simulink subsystem "unreal_cosim"  (R2026a)
settings: Solver=VariableStepAuto
undefined symbols (not defined in the file): M_WorldToUCS, S, scene_config, Sim3dSensor
libraries: sim3dlib x32, visionsinks x4, sim3dcameralib x4, dspvision x4
PreSaveFcn:
  | deconfigure_scene(bdroot)
  | defaultToFileBlockNames(bdroot);
settings Model: Creator=kjhaydon  LastModifiedBy=kjhaydon

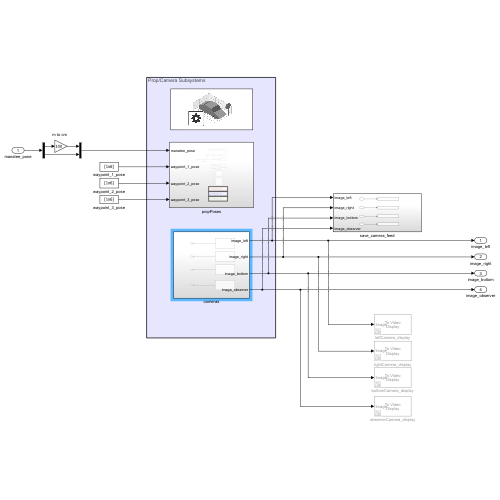
[thumbnail: Simulink's stored preview of the top-level diagram]
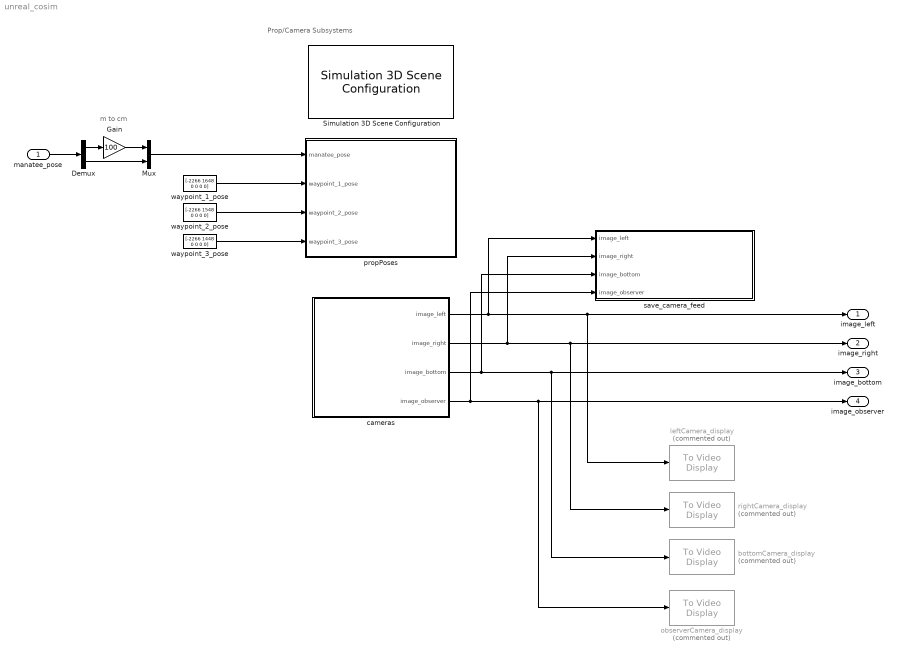
== system unreal_cosim ==
  note: m to cm
  note: Prop/Camera Subsystems
  manatee_pose : Inport  SampleTime=S.dt_sample
  Demux : Demux  Outputs=2
  Gain : Gain  Gain=100
  Mux : Mux  Inputs=2
  Simulation 3D Scene Configuration : sim3dlib/Simulation 3D Scene Configuration  Priority=0  ProjectFormat=Unreal Executable  SceneDesc=Empty scene  ProjectName=C:\Users\kjhaydon\Documents\GitHub\controls-2027\src\unreal_executables\EllingtonPoolSim_2_beta\Windows\EllingtonPoolSim2.exe  ScenePath=/Game/Olympic_Pool_Course  UEProjPath=C:\Users\Liam\OneDrive\Documents\Unreal Projects\EllingtonPoolSim2\EllingtonPoolSim2.uproject  EnableOpenDRIVE=off  vehTagList={'Custom';'Scene Origin'}  vehTag=Scene Origin  AttachedCameraRelativeTranslation=[0 0 0]  FreeCameraDefaultInitialTranslation=[-6, 0, 2]  AttachedCameraRelativeRotation=[0, -15, 0]  FreeCameraDefaultInitialRotation=[0, -15, 0]  ViewpointName=Custom  FreeCameraInitialTranslation=[0, 0, 0]  FreeCameraInitialRotation=[0, 0, 0]  OpVisEn=off  Ts=S.dt_sample  EnableWindow=off  EnableRemoteAccess=off  SimulationMode=CoSimulation  SimulateUsing=Interpreted execution  EnableAnimationRecording=off  OverrideDefaultRecording=off  AnimationRecordingFileName=sim3dAnimation.mat  AnimationRecordingInterval=[0 inf]  EnableWeather=off  SunAzimuth=90  SunAltitude=40.0  EnableGeospatialSun=off  Latitude=0  Longitude=0  Date=2023-01-01  Time=10:30:00  GeoTimeZone=-5.0  SunDaylightSaving=off  wind=1  clouds=10  EnableVolumetricClouds=off  CloudCoverage=0  CloudAltitude=6  fog=0  rain=0  RaindropsEffect=off  SnowDensity=0  EnableGeospatial=off  TilesetSource=Earth terrain  UseTrueOrigin=off  OriginHeight=200  OriginLatitude=40.744652  OriginLongitude=-73.988864  MapStyle=Aerial  AdditionalAssetIDs=[]  UseAdvancedSunSky=off  SolarTime=11  TimeZone=-5  Day=21  Month=9  Year=2022  UseDaylightSavingTime=on  DSTStartDay=10  DSTStartMonth=3  DSTEndDay=3  DSTEndMonth=11  DSTSwitchHour=2  sensorTag=MainCamera2  sensorId=2  sensorName=MainCamera2  mountLoc=Origin  offsetFlag=off  tmountOffset=[0, 0, 0]  rmountOffset=[0, 0, 0]  HorizontalResolution=1280  VerticalResolution=720  HorizontalFOV=60  mountPoint=[0 0 0]  mountOrientation=[0 0 0]  aMode=5  ID=2  GeoTrigger=Inactive  ViewNameList={'Custom'}  ViewTranslationList={'[0 0 0]'}  ViewRotationList={'[0 0 0]'}
      settings: LibrarySourceBlock=sl3dlib/Simulation 3D/Environment/Simulation 3D Scene Configuration
  bottomCamera_display : visionsinks/To Video Display  Commented=on  windowSizeMode=Normal  openAtMdlStart=off  fullScreen=off  videoWindowX=536805376  videoWindowY=536805376  saveWindowSize=off  videoWindowWidth=1491  videoWindowHeight=834  inputColorFormat=RGB  inputType=Obsolete  imagePorts=One multidimensional signal  OutputDevice=On-screen video monitor  dataOrg=Column-major  isWindowOpen=off
  cameras : Subsystem
  leftCamera_display : visionsinks/To Video Display  Commented=on  windowSizeMode=Normal  openAtMdlStart=on  fullScreen=off  videoWindowX=536805376  videoWindowY=536805376  saveWindowSize=off  videoWindowWidth=1491  videoWindowHeight=834  inputColorFormat=RGB  inputType=Obsolete  imagePorts=One multidimensional signal  OutputDevice=On-screen video monitor  dataOrg=Column-major  isWindowOpen=off
  observerCamera_display : visionsinks/To Video Display  Commented=on  windowSizeMode=Normal  openAtMdlStart=on  fullScreen=off  videoWindowX=536805376  videoWindowY=536805376  saveWindowSize=off  videoWindowWidth=1491  videoWindowHeight=834  inputColorFormat=RGB  inputType=Obsolete  imagePorts=One multidimensional signal  OutputDevice=On-screen video monitor  dataOrg=Column-major  isWindowOpen=off
  propPoses : Subsystem  Priority=1
  rightCamera_display : visionsinks/To Video Display  Commented=on  windowSizeMode=Normal  openAtMdlStart=on  fullScreen=off  videoWindowX=536805376  videoWindowY=536805376  saveWindowSize=off  videoWindowWidth=1491  videoWindowHeight=834  inputColorFormat=RGB  inputType=Obsolete  imagePorts=One multidimensional signal  OutputDevice=On-screen video monitor  dataOrg=Column-major  isWindowOpen=off
  save_camera_feed : Subsystem
  waypoint_1_pose : Constant  Value=[-2266 1648 0 0 0 0]
  waypoint_2_pose : Constant  Value=[-2266 1548 0 0 0 0]
  waypoint_3_pose : Constant  Value=[-2266 1448 0 0 0 0]
  image_left : Outport
  image_right : Outport  Port=2
  image_bottom : Outport  Port=3
  image_observer : Outport  Port=4
  wires:
  waypoint_3_pose/1 -> propPoses/4(waypoint_3_pose)
  waypoint_2_pose/1 -> propPoses/3(waypoint_2_pose)
  waypoint_1_pose/1 -> propPoses/2(waypoint_1_pose)
  Demux/1 -> Gain/1
  Gain/1 -> Mux/1
  Demux/2 -> Mux/2
  manatee_pose/1 -> Demux/1
  Mux/1 -> propPoses/1(manatee_pose)
  cameras/4(image_observer) -> save_camera_feed/4(image_observer), observerCamera_display/1, image_observer/1
  cameras/1(image_left) -> save_camera_feed/1(image_left), leftCamera_display/1, image_left/1
  cameras/2(image_right) -> rightCamera_display/1, image_right/1, save_camera_feed/2(image_right)
  cameras/3(image_bottom) -> bottomCamera_display/1, image_bottom/1, save_camera_feed/3(image_bottom)

== system unreal_cosim/cameras ==
  Bottom Camera ID:1 : sim3dcameralib/Simulation 3D Camera  Priority=1  sensorTag=Sim3dSensor�  sensorId=1  sensorName=Sim3dSensor�  vehTagList={'Custom ...';'Scene Origin'}  vehTag=Scene Origin  CoordinateSystem=Default  mountLoc=Origin  offsetFlag=on  tmountOffset=scene_config.cameras.bottomCamera.Position  extTmount=off  rmountOffset=scene_config.cameras.bottomCamera.Orientation  extRmount=off  FocalLength=scene_config.cameras.bottomCamera.FocalLength  OpticalCenter=scene_config.cameras.bottomCamera.OpticalCenter  ImageSize=scene_config.cameras.bottomCamera.ImageSize  RadialDistortion=scene_config.cameras.bottomCamera.RadialDistortion  TangentialDistortion=scene_config.cameras.bottomCamera.TangentialDistortion  SensorSkew=0  VisualizeFieldOfView=off  FieldOfViewRange=61  DepthOutportEnabled=off  SemanticOutportEnabled=off  TransformOutportEnabled=off  SampleTime=S.dt_sample  mountPoint=[0.23 0 -0.08]  mountOrientation=[0 -90 0]  aMode=5  ID=1
      settings: LibrarySourceBlock=sl3dlib/Simulation 3D/Sensors/Simulation 3D Camera
  Left Camera ID:2 : sim3dcameralib/Simulation 3D Camera  Priority=1  sensorTag=Sim3dSensor�  sensorId=2  sensorName=Sim3dSensor�  vehTagList={'Custom ...';'Scene Origin'}  vehTag=Scene Origin  CoordinateSystem=Default  mountLoc=Origin  offsetFlag=on  tmountOffset=scene_config.cameras.leftCamera.Position  extTmount=off  rmountOffset=scene_config.cameras.leftCamera.Orientation  extRmount=off  FocalLength=scene_config.cameras.leftCamera.FocalLength  OpticalCenter=scene_config.cameras.leftCamera.OpticalCenter  ImageSize=scene_config.cameras.leftCamera.ImageSize  RadialDistortion=scene_config.cameras.leftCamera.RadialDistortion  TangentialDistortion=scene_config.cameras.leftCamera.TangentialDistortion  SensorSkew=0  VisualizeFieldOfView=off  FieldOfViewRange=61  DepthOutportEnabled=off  SemanticOutportEnabled=off  TransformOutportEnabled=off  SampleTime=S.dt_sample  mountPoint=[0.38 -0.024 0.14]  mountOrientation=[0 0 0]  aMode=5  ID=2
      settings: LibrarySourceBlock=sl3dlib/Simulation 3D/Sensors/Simulation 3D Camera
  Observer Camera ID:4 : sim3dcameralib/Simulation 3D Camera  Priority=1  sensorTag=Sim3dSensor�  sensorId=4  sensorName=Sim3dSensor�  vehTagList={'Custom ...';'Scene Origin'}  vehTag=Scene Origin  CoordinateSystem=Default  mountLoc=Origin  offsetFlag=on  tmountOffset=scene_config.cameras.observerCamera.Position  extTmount=off  rmountOffset=scene_config.cameras.observerCamera.Orientation  extRmount=off  FocalLength=scene_config.cameras.observerCamera.FocalLength  OpticalCenter=scene_config.cameras.observerCamera.OpticalCenter  ImageSize=scene_config.cameras.observerCamera.ImageSize  RadialDistortion=scene_config.cameras.observerCamera.RadialDistortion  TangentialDistortion=scene_config.cameras.observerCamera.TangentialDistortion  SensorSkew=0  VisualizeFieldOfView=off  FieldOfViewRange=61  DepthOutportEnabled=off  SemanticOutportEnabled=off  TransformOutportEnabled=off  SampleTime=S.dt_sample  mountPoint=[0 0 0]  mountOrientation=[0 0 0]  aMode=5  ID=4
      settings: LibrarySourceBlock=sl3dlib/Simulation 3D/Sensors/Simulation 3D Camera
  Right Camera ID:3 : sim3dcameralib/Simulation 3D Camera  Priority=1  sensorTag=Sim3dSensor�  sensorId=3  sensorName=Sim3dSensor�  vehTagList={'Custom ...';'Scene Origin'}  vehTag=Scene Origin  CoordinateSystem=Default  mountLoc=Origin  offsetFlag=on  tmountOffset=scene_config.cameras.rightCamera.Position  extTmount=off  rmountOffset=scene_config.cameras.rightCamera.Orientation  extRmount=off  FocalLength=scene_config.cameras.rightCamera.FocalLength  OpticalCenter=scene_config.cameras.rightCamera.OpticalCenter  ImageSize=scene_config.cameras.rightCamera.ImageSize  RadialDistortion=scene_config.cameras.rightCamera.RadialDistortion  TangentialDistortion=scene_config.cameras.rightCamera.TangentialDistortion  SensorSkew=0  VisualizeFieldOfView=off  FieldOfViewRange=61  DepthOutportEnabled=off  SemanticOutportEnabled=off  TransformOutportEnabled=off  SampleTime=S.dt_sample  mountPoint=[0.38 0.024 0.14]  mountOrientation=[0 0 0]  aMode=5  ID=3
      settings: LibrarySourceBlock=sl3dlib/Simulation 3D/Sensors/Simulation 3D Camera
  image_left : Outport
  image_right : Outport  Port=2
  image_bottom : Outport  Port=3
  image_observer : Outport  Port=4
  wires:
  Observer Camera ID:4/1 -> image_observer/1
  Bottom Camera ID:1/1 -> image_bottom/1
  Right Camera ID:3/1 -> image_right/1
  Left Camera ID:2/1 -> image_left/1

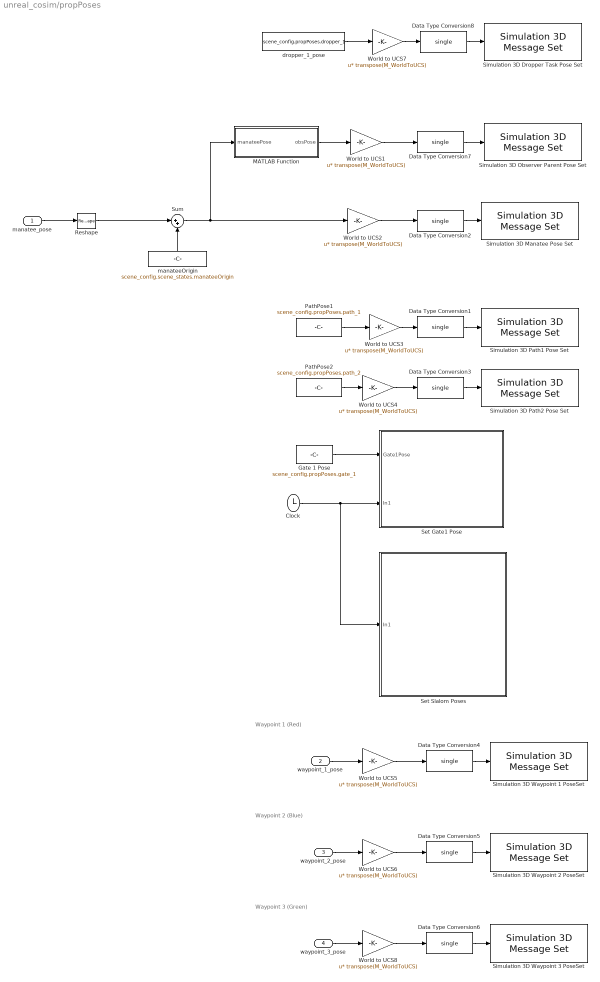
== system unreal_cosim/propPoses ==
  note: Waypoint 3 (Green)
  note: Waypoint 2 (Blue)
  note: Waypoint 1 (Red)
  manatee_pose : Inport
  waypoint_1_pose : Inport  Port=2
  waypoint_2_pose : Inport  Port=3
  waypoint_3_pose : Inport  Port=4
  Clock : Clock
      settings: Decimation=S.dt_sample/S.dt_sim
  Data Type Conversion{1..8} (8 alike) : DataTypeConversion  OutDataTypeStr=single  SaturateOnIntegerOverflow=off  RndMeth=Floor
  Gate 1 Pose : Constant  Value=scene_config.propPoses.gate_1
  MATLAB Function : MATLAB Function  TreatAsAtomicUnit=on
  PathPose1 : Constant  Value=scene_config.propPoses.path_1
  PathPose2 : Constant  Value=scene_config.propPoses.path_2
  Reshape : Reshape  OutputDimensionality=Row vector (2-D)
  Set Gate1 Pose : Subsystem
  Set Slalom Poses : Subsystem
  Simulation 3D Dropper Task Pose Set : sim3dlib/Simulation 3D Message Set  Priority=-1  SigName=DropperTask1PoseSet  Ts=S.dt_sample  aMode=0
      settings: LibrarySourceBlock=aerolibsim3d/Simulation 3D Message Set
  Simulation 3D Manatee Pose Set : sim3dlib/Simulation 3D Message Set  Priority=-1  SigName=ManateePoseSet  Ts=S.dt_sample  aMode=0
      settings: LibrarySourceBlock=aerolibsim3d/Simulation 3D Message Set
  Simulation 3D Observer Parent Pose Set : sim3dlib/Simulation 3D Message Set  Priority=-1  SigName=ParentPoseSet  Ts=S.dt_sample  aMode=0
      settings: LibrarySourceBlock=aerolibsim3d/Simulation 3D Message Set
  Simulation 3D Path1 Pose Set : sim3dlib/Simulation 3D Message Set  Priority=-1  SigName=Path1PoseSet  Ts=S.dt_sample  aMode=0
      settings: LibrarySourceBlock=aerolibsim3d/Simulation 3D Message Set
  Simulation 3D Path2 Pose Set : sim3dlib/Simulation 3D Message Set  Priority=-1  SigName=Path2PoseSet  Ts=S.dt_sample  aMode=0
      settings: LibrarySourceBlock=aerolibsim3d/Simulation 3D Message Set
  Simulation 3D Waypoint 1 PoseSet : sim3dlib/Simulation 3D Message Set  Priority=-1  SigName=Waypoint1PoseSet  Ts=S.dt_sample  aMode=0
      settings: LibrarySourceBlock=aerolibsim3d/Simulation 3D Message Set
  Simulation 3D Waypoint 2 PoseSet : sim3dlib/Simulation 3D Message Set  Priority=-1  SigName=Waypoint2PoseSet  Ts=S.dt_sample  aMode=0
      settings: LibrarySourceBlock=aerolibsim3d/Simulation 3D Message Set
  Simulation 3D Waypoint 3 PoseSet : sim3dlib/Simulation 3D Message Set  Priority=-1  SigName=Waypoint3PoseSet  Ts=S.dt_sample  aMode=0
      settings: LibrarySourceBlock=aerolibsim3d/Simulation 3D Message Set
  Sum : Sum  Inputs=|++
  World to UCS{1..8} (8 alike) : Gain  Gain=transpose(M_WorldToUCS)  Multiplication=Matrix(u*K)
  dropper_1_pose : Constant  Value=scene_config.propPoses.dropper_1
  manateeOrigin : Constant  Value=scene_config.scene_states.manateeOrigin
  wires:
  Reshape/1 -> Sum/1
  waypoint_3_pose/1 -> World to UCS8/1
  dropper_1_pose/1 -> World to UCS7/1
  World to UCS7/1 -> Data Type Conversion8/1
  Data Type Conversion8/1 -> Simulation 3D Dropper Task Pose Set/1
  MATLAB Function/1(obsPose) -> World to UCS1/1
  World to UCS1/1 -> Data Type Conversion7/1
  Data Type Conversion7/1 -> Simulation 3D Observer Parent Pose Set/1
  manateeOrigin/1 -> Sum/2
  Sum/1 -> MATLAB Function/1(manateePose), World to UCS2/1
  manatee_pose/1 -> Reshape/1
  Data Type Conversion6/1 -> Simulation 3D Waypoint 3 PoseSet/1
  World to UCS8/1 -> Data Type Conversion6/1
  World to UCS6/1 -> Data Type Conversion5/1
  Data Type Conversion5/1 -> Simulation 3D Waypoint 2 PoseSet/1
  waypoint_2_pose/1 -> World to UCS6/1
  World to UCS5/1 -> Data Type Conversion4/1
  Data Type Conversion4/1 -> Simulation 3D Waypoint 1 PoseSet/1
  waypoint_1_pose/1 -> World to UCS5/1
  World to UCS2/1 -> Data Type Conversion2/1
  Clock/1 -> Set Gate1 Pose/2(In1), Set Slalom Poses/1(In1)
  PathPose2/1 -> World to UCS4/1
  Data Type Conversion3/1 -> Simulation 3D Path2 Pose Set/1
  World to UCS4/1 -> Data Type Conversion3/1
  PathPose1/1 -> World to UCS3/1
  Data Type Conversion1/1 -> Simulation 3D Path1 Pose Set/1
  World to UCS3/1 -> Data Type Conversion1/1
  Data Type Conversion2/1 -> Simulation 3D Manatee Pose Set/1
  Gate 1 Pose/1 -> Set Gate1 Pose/1(Gate1Pose)

== system unreal_cosim/save_camera_feed ==
  image_left : Inport
  image_right : Inport  Port=2
  image_bottom : Inport  Port=3
  image_observer : Inport  Port=4
  bottomCamera_save : dspvision/To Multimedia File  Commented=on  outputFilename=default  streamSelection=Video only  videoCompressor=None (uncompressed)  audioCompressor=None (uncompressed)  imagePorts=One multidimensional signal  fileType=MPEG4  audioDatatype=16-bit integer  fourcc=RGB  audioBitRate=128  audioQuality=75  videoQuality=75  mj2000CompFactor=10
      settings: LibrarySourceBlock=audiosinks/To Multimedia File
  leftCamera_save : dspvision/To Multimedia File  Commented=on  outputFilename=default  streamSelection=Video only  videoCompressor=None (uncompressed)  audioCompressor=None (uncompressed)  imagePorts=One multidimensional signal  fileType=MPEG4  audioDatatype=16-bit integer  fourcc=RGB  audioBitRate=128  audioQuality=75  videoQuality=75  mj2000CompFactor=10
      settings: LibrarySourceBlock=audiosinks/To Multimedia File
  observerCamera_save : dspvision/To Multimedia File  Commented=on  outputFilename=default  streamSelection=Video only  videoCompressor=None (uncompressed)  audioCompressor=None (uncompressed)  imagePorts=One multidimensional signal  fileType=MPEG4  audioDatatype=16-bit integer  fourcc=RGB  audioBitRate=128  audioQuality=75  videoQuality=75  mj2000CompFactor=10
      settings: LibrarySourceBlock=audiosinks/To Multimedia File
  rightCamera_save : dspvision/To Multimedia File  Commented=on  outputFilename=default  streamSelection=Video only  videoCompressor=None (uncompressed)  audioCompressor=None (uncompressed)  imagePorts=One multidimensional signal  fileType=MPEG4  audioDatatype=16-bit integer  fourcc=RGB  audioBitRate=128  audioQuality=75  videoQuality=75  mj2000CompFactor=10
      settings: LibrarySourceBlock=audiosinks/To Multimedia File
  wires:
  image_left/1 -> leftCamera_save/1
  image_observer/1 -> observerCamera_save/1
  image_bottom/1 -> bottomCamera_save/1
  image_right/1 -> rightCamera_save/1

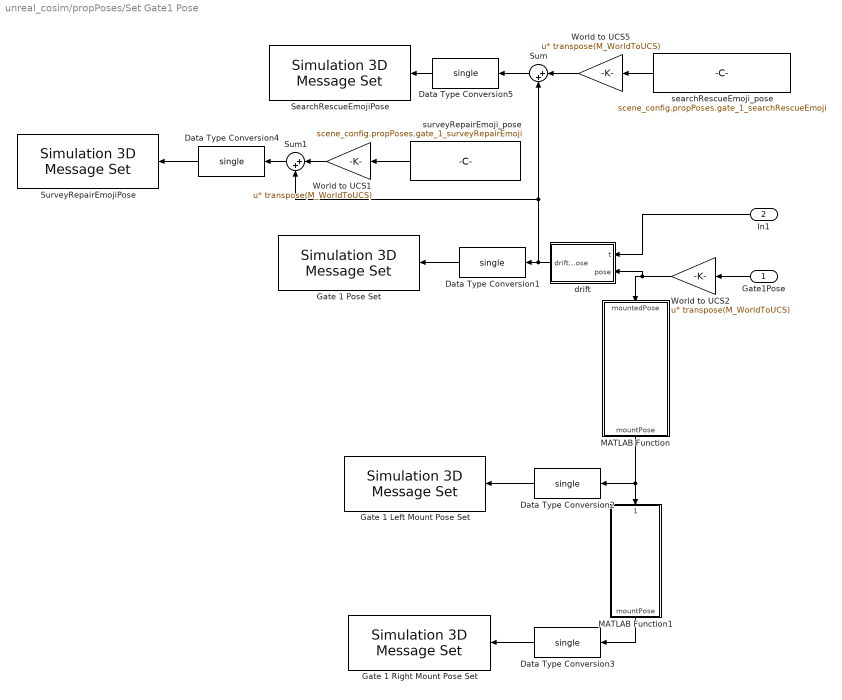
== system unreal_cosim/propPoses/Set Gate1 Pose ==
  Gate1Pose : Inport
  In1 : Inport  Port=2
  Data Type Conversion{1..5} (5 alike) : DataTypeConversion  OutDataTypeStr=single  SaturateOnIntegerOverflow=off  RndMeth=Floor
  Gate 1 Left Mount Pose Set : sim3dlib/Simulation 3D Message Set  Priority=-1  SigName=Gate1LeftMountPoseSet  Ts=S.dt_sample  aMode=0
      settings: LibrarySourceBlock=aerolibsim3d/Simulation 3D Message Set
  Gate 1 Pose Set : sim3dlib/Simulation 3D Message Set  Priority=-1  SigName=Gate1PoseSet  Ts=S.dt_sample  aMode=0
      settings: LibrarySourceBlock=aerolibsim3d/Simulation 3D Message Set
  Gate 1 Right Mount Pose Set : sim3dlib/Simulation 3D Message Set  Priority=-1  SigName=Gate1RightMountPoseSet  Ts=S.dt_sample  aMode=0
      settings: LibrarySourceBlock=aerolibsim3d/Simulation 3D Message Set
  MATLAB Function : MATLAB Function  TreatAsAtomicUnit=on
  MATLAB Function1 : MATLAB Function  TreatAsAtomicUnit=on
  SearchRescueEmojiPose : sim3dlib/Simulation 3D Message Set  Priority=-1  SigName=SearchRescueEmojiPoseSet  Ts=S.dt_sample  aMode=0
      settings: LibrarySourceBlock=aerolibsim3d/Simulation 3D Message Set
  Sum : Sum  Inputs=|++
  Sum1 : Sum  Inputs=|++
  SurveyRepairEmojiPose : sim3dlib/Simulation 3D Message Set  Priority=-1  SigName=SurveyRepairEmojiPoseSet  Ts=S.dt_sample  aMode=0
      settings: LibrarySourceBlock=aerolibsim3d/Simulation 3D Message Set
  World to UCS1 : Gain  Gain=transpose(M_WorldToUCS)  Multiplication=Matrix(u*K)
  World to UCS2 : Gain  Gain=transpose(M_WorldToUCS)  Multiplication=Matrix(u*K)
  World to UCS5 : Gain  Gain=transpose(M_WorldToUCS)  Multiplication=Matrix(u*K)
  drift : MATLAB Function  TreatAsAtomicUnit=on
  searchRescueEmoji_pose : Constant  Value=scene_config.propPoses.gate_1_searchRescueEmoji
  surveyRepairEmoji_pose : Constant  Value=scene_config.propPoses.gate_1_surveyRepairEmoji
  wires:
  drift/1(driftPose) -> Data Type Conversion1/1, Sum/2, Sum1/2
  In1/1 -> drift/1(t)
  Sum1/1 -> Data Type Conversion4/1
  World to UCS1/1 -> Sum1/1
  World to UCS5/1 -> Sum/1
  Sum/1 -> Data Type Conversion5/1
  searchRescueEmoji_pose/1 -> World to UCS5/1
  Data Type Conversion5/1 -> SearchRescueEmojiPose/1
  surveyRepairEmoji_pose/1 -> World to UCS1/1
  Data Type Conversion4/1 -> SurveyRepairEmojiPose/1
  MATLAB Function1/1(mountPose) -> Data Type Conversion3/1
  World to UCS2/1 -> MATLAB Function/1(mountedPose), drift/2(pose)
  Data Type Conversion1/1 -> Gate 1 Pose Set/1
  Data Type Conversion3/1 -> Gate 1 Right Mount Pose Set/1
  Data Type Conversion2/1 -> Gate 1 Left Mount Pose Set/1
  MATLAB Function/1(mountPose) -> MATLAB Function1/1(leftMountPose), Data Type Conversion2/1
  Gate1Pose/1 -> World to UCS2/1

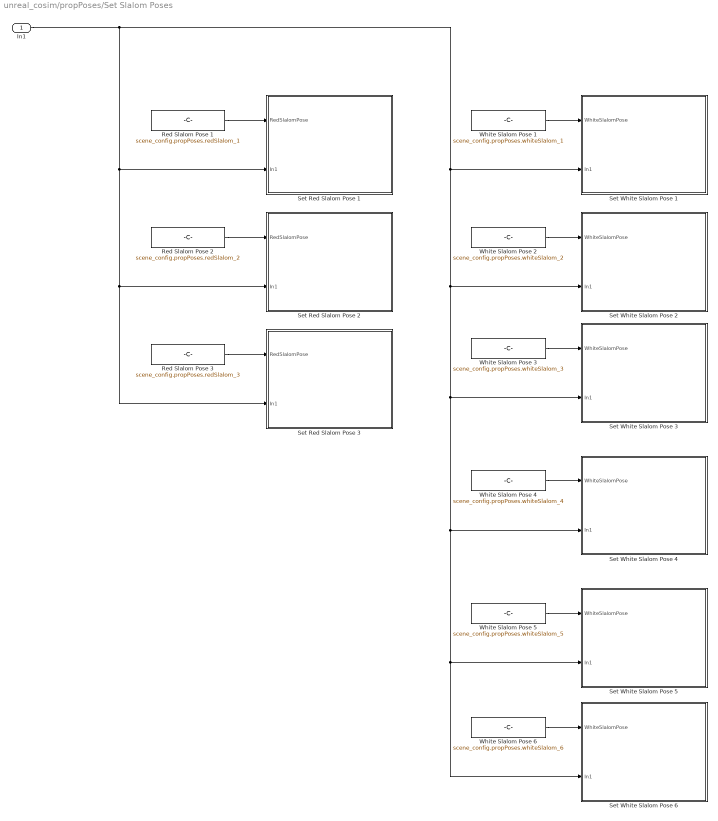
== system unreal_cosim/propPoses/Set Slalom Poses ==
  In1 : Inport
  Red Slalom Pose 1 : Constant  Value=scene_config.propPoses.redSlalom_1
  Red Slalom Pose 2 : Constant  Value=scene_config.propPoses.redSlalom_2
  Red Slalom Pose 3 : Constant  Value=scene_config.propPoses.redSlalom_3
  Set Red Slalom Pose 1 : Subsystem
  Set Red Slalom Pose 2 : Subsystem
  Set Red Slalom Pose 3 : Subsystem
  Set White Slalom Pose 1 : Subsystem
  Set White Slalom Pose 2 : Subsystem
  Set White Slalom Pose 3 : Subsystem
  Set White Slalom Pose 4 : Subsystem
  Set White Slalom Pose 5 : Subsystem
  Set White Slalom Pose 6 : Subsystem
  White Slalom Pose 1 : Constant  Value=scene_config.propPoses.whiteSlalom_1
  White Slalom Pose 2 : Constant  Value=scene_config.propPoses.whiteSlalom_2
  White Slalom Pose 3 : Constant  Value=scene_config.propPoses.whiteSlalom_3
  White Slalom Pose 4 : Constant  Value=scene_config.propPoses.whiteSlalom_4
  White Slalom Pose 5 : Constant  Value=scene_config.propPoses.whiteSlalom_5
  White Slalom Pose 6 : Constant  Value=scene_config.propPoses.whiteSlalom_6
  wires:
  In1/1 -> Set White Slalom Pose 1/2(In1), Set White Slalom Pose 2/2(In1), Set White Slalom Pose 3/2(In1), Set White Slalom Pose 4/2(In1), Set White Slalom Pose 5/2(In1), Set White Slalom Pose 6/2(In1), Set Red Slalom Pose 1/2(In1), Set Red Slalom Pose 2/2(In1), Set Red Slalom Pose 3/2(In1)
  White Slalom Pose 6/1 -> Set White Slalom Pose 6/1(WhiteSlalomPose)
  White Slalom Pose 5/1 -> Set White Slalom Pose 5/1(WhiteSlalomPose)
  White Slalom Pose 4/1 -> Set White Slalom Pose 4/1(WhiteSlalomPose)
  White Slalom Pose 3/1 -> Set White Slalom Pose 3/1(WhiteSlalomPose)
  White Slalom Pose 2/1 -> Set White Slalom Pose 2/1(WhiteSlalomPose)
  White Slalom Pose 1/1 -> Set White Slalom Pose 1/1(WhiteSlalomPose)
  Red Slalom Pose 3/1 -> Set Red Slalom Pose 3/1(RedSlalomPose)
  Red Slalom Pose 2/1 -> Set Red Slalom Pose 2/1(RedSlalomPose)
  Red Slalom Pose 1/1 -> Set Red Slalom Pose 1/1(RedSlalomPose)

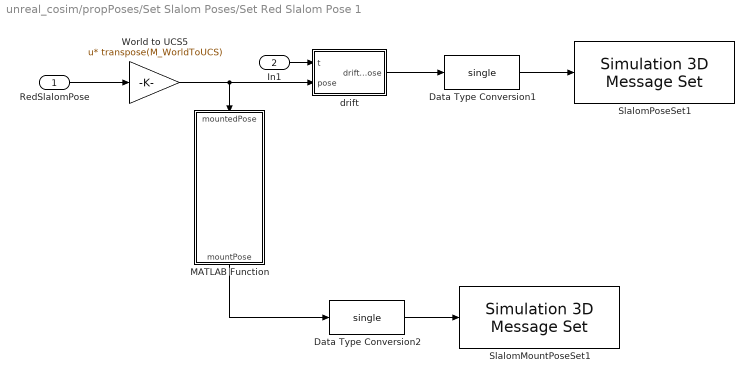
== system unreal_cosim/propPoses/Set Slalom Poses/Set Red Slalom Pose 1 ==
  RedSlalomPose : Inport
  In1 : Inport  Port=2
  Data Type Conversion1 : DataTypeConversion  OutDataTypeStr=single  SaturateOnIntegerOverflow=off  RndMeth=Floor
  Data Type Conversion2 : DataTypeConversion  OutDataTypeStr=single  SaturateOnIntegerOverflow=off  RndMeth=Floor
  MATLAB Function : MATLAB Function  TreatAsAtomicUnit=on
  SlalomMountPoseSet1 : sim3dlib/Simulation 3D Message Set  Priority=-1  SigName=RedSlalom1MountPoseSet  Ts=S.dt_sample  aMode=0
      settings: LibrarySourceBlock=aerolibsim3d/Simulation 3D Message Set
  SlalomPoseSet1 : sim3dlib/Simulation 3D Message Set  Priority=-1  SigName=RedSlalom1PoseSet  Ts=S.dt_sample  aMode=0
      settings: LibrarySourceBlock=aerolibsim3d/Simulation 3D Message Set
  World to UCS5 : Gain  Gain=transpose(M_WorldToUCS)  Multiplication=Matrix(u*K)
  drift : MATLAB Function  TreatAsAtomicUnit=on
  wires:
  In1/1 -> drift/1(t)
  drift/1(driftPose) -> Data Type Conversion1/1
  World to UCS5/1 -> MATLAB Function/1(mountedPose), drift/2(pose)
  Data Type Conversion1/1 -> SlalomPoseSet1/1
  Data Type Conversion2/1 -> SlalomMountPoseSet1/1
  MATLAB Function/1(mountPose) -> Data Type Conversion2/1
  RedSlalomPose/1 -> World to UCS5/1

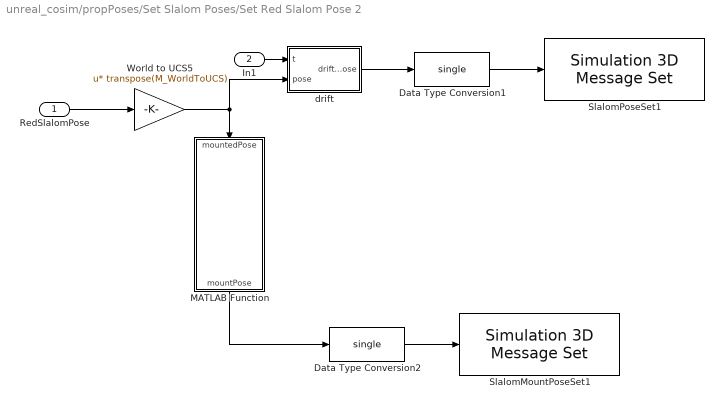
== system unreal_cosim/propPoses/Set Slalom Poses/Set Red Slalom Pose 2 ==
  RedSlalomPose : Inport
  In1 : Inport  Port=2
  Data Type Conversion1 : DataTypeConversion  OutDataTypeStr=single  SaturateOnIntegerOverflow=off  RndMeth=Floor
  Data Type Conversion2 : DataTypeConversion  OutDataTypeStr=single  SaturateOnIntegerOverflow=off  RndMeth=Floor
  MATLAB Function : MATLAB Function  TreatAsAtomicUnit=on
  SlalomMountPoseSet1 : sim3dlib/Simulation 3D Message Set  Priority=-1  SigName=RedSlalom2MountPoseSet  Ts=S.dt_sample  aMode=0
      settings: LibrarySourceBlock=aerolibsim3d/Simulation 3D Message Set
  SlalomPoseSet1 : sim3dlib/Simulation 3D Message Set  Priority=-1  SigName=RedSlalom2PoseSet  Ts=S.dt_sample  aMode=0
      settings: LibrarySourceBlock=aerolibsim3d/Simulation 3D Message Set
  World to UCS5 : Gain  Gain=transpose(M_WorldToUCS)  Multiplication=Matrix(u*K)
  drift : MATLAB Function  TreatAsAtomicUnit=on
  wires:
  drift/1(driftPose) -> Data Type Conversion1/1
  In1/1 -> drift/1(t)
  World to UCS5/1 -> drift/2(pose), MATLAB Function/1(mountedPose)
  Data Type Conversion1/1 -> SlalomPoseSet1/1
  Data Type Conversion2/1 -> SlalomMountPoseSet1/1
  MATLAB Function/1(mountPose) -> Data Type Conversion2/1
  RedSlalomPose/1 -> World to UCS5/1

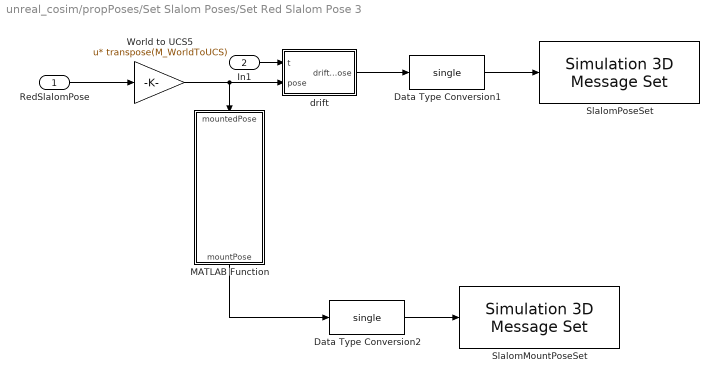
== system unreal_cosim/propPoses/Set Slalom Poses/Set Red Slalom Pose 3 ==
  RedSlalomPose : Inport
  In1 : Inport  Port=2
  Data Type Conversion1 : DataTypeConversion  OutDataTypeStr=single  SaturateOnIntegerOverflow=off  RndMeth=Floor
  Data Type Conversion2 : DataTypeConversion  OutDataTypeStr=single  SaturateOnIntegerOverflow=off  RndMeth=Floor
  MATLAB Function : MATLAB Function  TreatAsAtomicUnit=on
  SlalomMountPoseSet : sim3dlib/Simulation 3D Message Set  Priority=-1  SigName=RedSlalom3MountPoseSet  Ts=S.dt_sample  aMode=0
      settings: LibrarySourceBlock=aerolibsim3d/Simulation 3D Message Set
  SlalomPoseSet : sim3dlib/Simulation 3D Message Set  Priority=-1  SigName=RedSlalom3PoseSet  Ts=S.dt_sample  aMode=0
      settings: LibrarySourceBlock=aerolibsim3d/Simulation 3D Message Set
  World to UCS5 : Gain  Gain=transpose(M_WorldToUCS)  Multiplication=Matrix(u*K)
  drift : MATLAB Function  TreatAsAtomicUnit=on
  wires:
  drift/1(driftPose) -> Data Type Conversion1/1
  In1/1 -> drift/1(t)
  World to UCS5/1 -> MATLAB Function/1(mountedPose), drift/2(pose)
  Data Type Conversion1/1 -> SlalomPoseSet/1
  Data Type Conversion2/1 -> SlalomMountPoseSet/1
  MATLAB Function/1(mountPose) -> Data Type Conversion2/1
  RedSlalomPose/1 -> World to UCS5/1

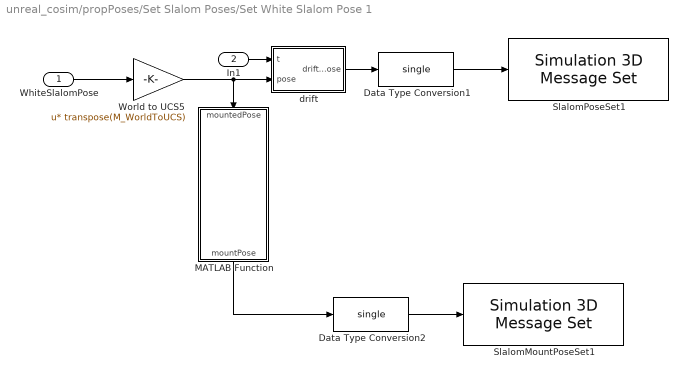
== system unreal_cosim/propPoses/Set Slalom Poses/Set White Slalom Pose 1 ==
  WhiteSlalomPose : Inport
  In1 : Inport  Port=2
  Data Type Conversion1 : DataTypeConversion  OutDataTypeStr=single  SaturateOnIntegerOverflow=off  RndMeth=Floor
  Data Type Conversion2 : DataTypeConversion  OutDataTypeStr=single  SaturateOnIntegerOverflow=off  RndMeth=Floor
  MATLAB Function : MATLAB Function  TreatAsAtomicUnit=on
  SlalomMountPoseSet1 : sim3dlib/Simulation 3D Message Set  Priority=-1  SigName=WhiteSlalom1MountPoseSet  Ts=S.dt_sample  aMode=0
      settings: LibrarySourceBlock=aerolibsim3d/Simulation 3D Message Set
  SlalomPoseSet1 : sim3dlib/Simulation 3D Message Set  Priority=-1  SigName=WhiteSlalom1PoseSet  Ts=S.dt_sample  aMode=0
      settings: LibrarySourceBlock=aerolibsim3d/Simulation 3D Message Set
  World to UCS5 : Gain  Gain=transpose(M_WorldToUCS)  Multiplication=Matrix(u*K)
  drift : MATLAB Function  TreatAsAtomicUnit=on
  wires:
  drift/1(driftPose) -> Data Type Conversion1/1
  In1/1 -> drift/1(t)
  World to UCS5/1 -> MATLAB Function/1(mountedPose), drift/2(pose)
  Data Type Conversion1/1 -> SlalomPoseSet1/1
  Data Type Conversion2/1 -> SlalomMountPoseSet1/1
  MATLAB Function/1(mountPose) -> Data Type Conversion2/1
  WhiteSlalomPose/1 -> World to UCS5/1

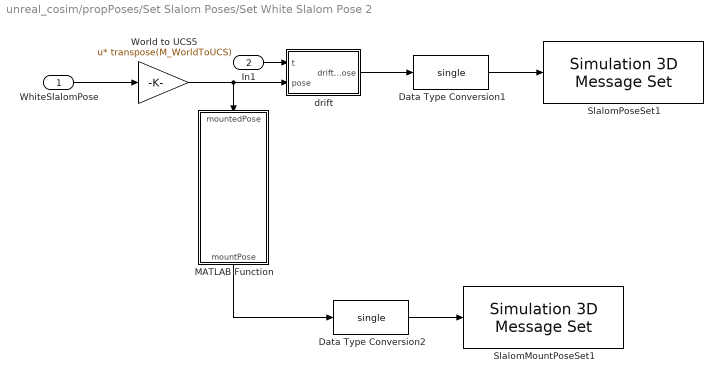
== system unreal_cosim/propPoses/Set Slalom Poses/Set White Slalom Pose 2 ==
  WhiteSlalomPose : Inport
  In1 : Inport  Port=2
  Data Type Conversion1 : DataTypeConversion  OutDataTypeStr=single  SaturateOnIntegerOverflow=off  RndMeth=Floor
  Data Type Conversion2 : DataTypeConversion  OutDataTypeStr=single  SaturateOnIntegerOverflow=off  RndMeth=Floor
  MATLAB Function : MATLAB Function  TreatAsAtomicUnit=on
  SlalomMountPoseSet1 : sim3dlib/Simulation 3D Message Set  Priority=-1  SigName=WhiteSlalom2MountPoseSet  Ts=S.dt_sample  aMode=0
      settings: LibrarySourceBlock=aerolibsim3d/Simulation 3D Message Set
  SlalomPoseSet1 : sim3dlib/Simulation 3D Message Set  Priority=-1  SigName=WhiteSlalom2PoseSet  Ts=S.dt_sample  aMode=0
      settings: LibrarySourceBlock=aerolibsim3d/Simulation 3D Message Set
  World to UCS5 : Gain  Gain=transpose(M_WorldToUCS)  Multiplication=Matrix(u*K)
  drift : MATLAB Function  TreatAsAtomicUnit=on
  wires:
  drift/1(driftPose) -> Data Type Conversion1/1
  In1/1 -> drift/1(t)
  World to UCS5/1 -> MATLAB Function/1(mountedPose), drift/2(pose)
  Data Type Conversion1/1 -> SlalomPoseSet1/1
  Data Type Conversion2/1 -> SlalomMountPoseSet1/1
  MATLAB Function/1(mountPose) -> Data Type Conversion2/1
  WhiteSlalomPose/1 -> World to UCS5/1

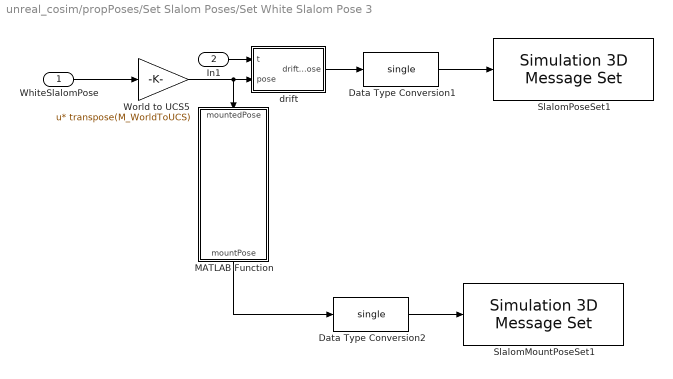
== system unreal_cosim/propPoses/Set Slalom Poses/Set White Slalom Pose 3 ==
  WhiteSlalomPose : Inport
  In1 : Inport  Port=2
  Data Type Conversion1 : DataTypeConversion  OutDataTypeStr=single  SaturateOnIntegerOverflow=off  RndMeth=Floor
  Data Type Conversion2 : DataTypeConversion  OutDataTypeStr=single  SaturateOnIntegerOverflow=off  RndMeth=Floor
  MATLAB Function : MATLAB Function  TreatAsAtomicUnit=on
  SlalomMountPoseSet1 : sim3dlib/Simulation 3D Message Set  Priority=-1  SigName=WhiteSlalom3MountPoseSet  Ts=S.dt_sample  aMode=0
      settings: LibrarySourceBlock=aerolibsim3d/Simulation 3D Message Set
  SlalomPoseSet1 : sim3dlib/Simulation 3D Message Set  Priority=-1  SigName=WhiteSlalom3PoseSet  Ts=S.dt_sample  aMode=0
      settings: LibrarySourceBlock=aerolibsim3d/Simulation 3D Message Set
  World to UCS5 : Gain  Gain=transpose(M_WorldToUCS)  Multiplication=Matrix(u*K)
  drift : MATLAB Function  TreatAsAtomicUnit=on
  wires:
  drift/1(driftPose) -> Data Type Conversion1/1
  In1/1 -> drift/1(t)
  World to UCS5/1 -> MATLAB Function/1(mountedPose), drift/2(pose)
  Data Type Conversion1/1 -> SlalomPoseSet1/1
  Data Type Conversion2/1 -> SlalomMountPoseSet1/1
  MATLAB Function/1(mountPose) -> Data Type Conversion2/1
  WhiteSlalomPose/1 -> World to UCS5/1

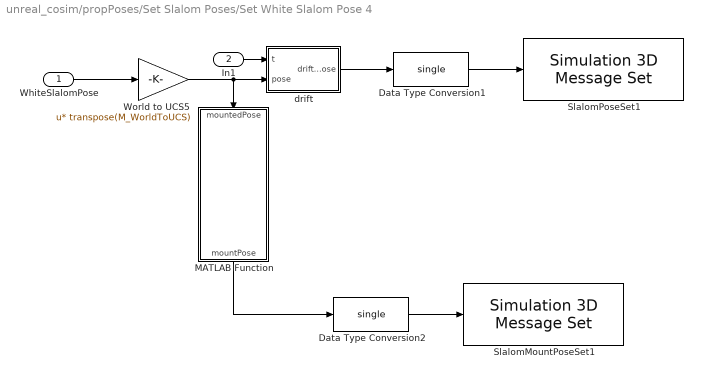
== system unreal_cosim/propPoses/Set Slalom Poses/Set White Slalom Pose 4 ==
  WhiteSlalomPose : Inport
  In1 : Inport  Port=2
  Data Type Conversion1 : DataTypeConversion  OutDataTypeStr=single  SaturateOnIntegerOverflow=off  RndMeth=Floor
  Data Type Conversion2 : DataTypeConversion  OutDataTypeStr=single  SaturateOnIntegerOverflow=off  RndMeth=Floor
  MATLAB Function : MATLAB Function  TreatAsAtomicUnit=on
  SlalomMountPoseSet1 : sim3dlib/Simulation 3D Message Set  Priority=-1  SigName=WhiteSlalom4MountPoseSet  Ts=S.dt_sample  aMode=0
      settings: LibrarySourceBlock=aerolibsim3d/Simulation 3D Message Set
  SlalomPoseSet1 : sim3dlib/Simulation 3D Message Set  Priority=-1  SigName=WhiteSlalom4PoseSet  Ts=S.dt_sample  aMode=0
      settings: LibrarySourceBlock=aerolibsim3d/Simulation 3D Message Set
  World to UCS5 : Gain  Gain=transpose(M_WorldToUCS)  Multiplication=Matrix(u*K)
  drift : MATLAB Function  TreatAsAtomicUnit=on
  wires:
  drift/1(driftPose) -> Data Type Conversion1/1
  In1/1 -> drift/1(t)
  World to UCS5/1 -> MATLAB Function/1(mountedPose), drift/2(pose)
  Data Type Conversion1/1 -> SlalomPoseSet1/1
  Data Type Conversion2/1 -> SlalomMountPoseSet1/1
  MATLAB Function/1(mountPose) -> Data Type Conversion2/1
  WhiteSlalomPose/1 -> World to UCS5/1

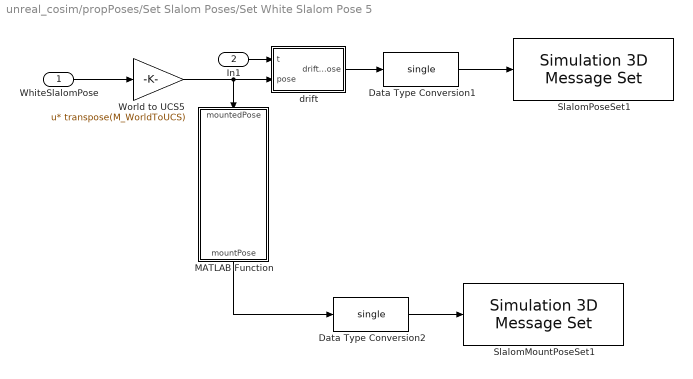
== system unreal_cosim/propPoses/Set Slalom Poses/Set White Slalom Pose 5 ==
  WhiteSlalomPose : Inport
  In1 : Inport  Port=2
  Data Type Conversion1 : DataTypeConversion  OutDataTypeStr=single  SaturateOnIntegerOverflow=off  RndMeth=Floor
  Data Type Conversion2 : DataTypeConversion  OutDataTypeStr=single  SaturateOnIntegerOverflow=off  RndMeth=Floor
  MATLAB Function : MATLAB Function  TreatAsAtomicUnit=on
  SlalomMountPoseSet1 : sim3dlib/Simulation 3D Message Set  Priority=-1  SigName=WhiteSlalom5MountPoseSet  Ts=S.dt_sample  aMode=0
      settings: LibrarySourceBlock=aerolibsim3d/Simulation 3D Message Set
  SlalomPoseSet1 : sim3dlib/Simulation 3D Message Set  Priority=-1  SigName=WhiteSlalom5PoseSet  Ts=S.dt_sample  aMode=0
      settings: LibrarySourceBlock=aerolibsim3d/Simulation 3D Message Set
  World to UCS5 : Gain  Gain=transpose(M_WorldToUCS)  Multiplication=Matrix(u*K)
  drift : MATLAB Function  TreatAsAtomicUnit=on
  wires:
  WhiteSlalomPose/1 -> World to UCS5/1
  drift/1(driftPose) -> Data Type Conversion1/1
  In1/1 -> drift/1(t)
  World to UCS5/1 -> MATLAB Function/1(mountedPose), drift/2(pose)
  Data Type Conversion1/1 -> SlalomPoseSet1/1
  Data Type Conversion2/1 -> SlalomMountPoseSet1/1
  MATLAB Function/1(mountPose) -> Data Type Conversion2/1

== system unreal_cosim/propPoses/Set Slalom Poses/Set White Slalom Pose 6 ==
  WhiteSlalomPose : Inport
  In1 : Inport  Port=2
  Data Type Conversion1 : DataTypeConversion  OutDataTypeStr=single  SaturateOnIntegerOverflow=off  RndMeth=Floor
  Data Type Conversion2 : DataTypeConversion  OutDataTypeStr=single  SaturateOnIntegerOverflow=off  RndMeth=Floor
  MATLAB Function : MATLAB Function  TreatAsAtomicUnit=on
  SlalomMountPoseSet1 : sim3dlib/Simulation 3D Message Set  Priority=-1  SigName=WhiteSlalom6MountPoseSet  Ts=S.dt_sample  aMode=0
      settings: LibrarySourceBlock=aerolibsim3d/Simulation 3D Message Set
  SlalomPoseSet1 : sim3dlib/Simulation 3D Message Set  Priority=-1  SigName=WhiteSlalom6PoseSet  Ts=S.dt_sample  aMode=0
      settings: LibrarySourceBlock=aerolibsim3d/Simulation 3D Message Set
  World to UCS5 : Gain  Gain=transpose(M_WorldToUCS)  Multiplication=Matrix(u*K)
  drift : MATLAB Function  TreatAsAtomicUnit=on
  wires:
  drift/1(driftPose) -> Data Type Conversion1/1
  In1/1 -> drift/1(t)
  World to UCS5/1 -> MATLAB Function/1(mountedPose), drift/2(pose)
  Data Type Conversion1/1 -> SlalomPoseSet1/1
  Data Type Conversion2/1 -> SlalomMountPoseSet1/1
  MATLAB Function/1(mountPose) -> Data Type Conversion2/1
  WhiteSlalomPose/1 -> World to UCS5/1

== matlab function unreal_cosim/propPoses/Set Gate1 Pose/MATLAB Function ==
  data: mountedPose input; mountPose output; ground_Z parameter
function mountPose = getMountPose(mountedPose, ground_Z)

mountPose = [mountedPose(1) mountedPose(2) (10 - ground_Z) 0 0 mountedPose(6)];

== matlab function unreal_cosim/propPoses/Set Slalom Poses/Set White Slalom Pose 2/drift ==
  data: t input; pose input; driftPose output
function driftPose = drift(t,pose)
driftPose = toDriftedCoordinates(pose,t);

== matlab function unreal_cosim/propPoses/Set Slalom Poses/Set White Slalom Pose 3/MATLAB Function ==
  data: mountedPose input; mountPose output; ground_Z parameter
function mountPose = getMountPose(mountedPose,ground_Z)

mountPose = [mountedPose(1) mountedPose(2) (10 - ground_Z) 0 0 mountedPose(6)];

== matlab function unreal_cosim/propPoses/Set Slalom Poses/Set White Slalom Pose 3/drift ==
  data: t input; pose input; driftPose output
function driftPose = drift(t,pose)
driftPose = toDriftedCoordinates(pose,t);

== matlab function unreal_cosim/propPoses/Set Slalom Poses/Set White Slalom Pose 4/MATLAB Function ==
  data: mountedPose input; mountPose output; ground_Z parameter
function mountPose = getMountPose(mountedPose,ground_Z)

mountPose = [mountedPose(1) mountedPose(2) (10 - ground_Z) 0 0 mountedPose(6)];

== matlab function unreal_cosim/propPoses/Set Slalom Poses/Set White Slalom Pose 4/drift ==
  data: t input; pose input; driftPose output
function driftPose = drift(t,pose)
driftPose = toDriftedCoordinates(pose,t);

== matlab function unreal_cosim/propPoses/Set Slalom Poses/Set White Slalom Pose 5/MATLAB Function ==
  data: mountedPose input; mountPose output; ground_Z parameter
function mountPose = getMountPose(mountedPose,ground_Z)

mountPose = [mountedPose(1) mountedPose(2) (10 - ground_Z) 0 0 mountedPose(6)];

== matlab function unreal_cosim/propPoses/Set Slalom Poses/Set White Slalom Pose 5/drift ==
  data: t input; pose input; driftPose output
function driftPose = drift(t,pose)
driftPose = toDriftedCoordinates(pose,t);

== matlab function unreal_cosim/propPoses/Set Slalom Poses/Set White Slalom Pose 6/MATLAB Function ==
  data: mountedPose input; mountPose output; ground_Z parameter
function mountPose = getMountPose(mountedPose,ground_Z)

mountPose = [mountedPose(1) mountedPose(2) (10 - ground_Z) 0 0 mountedPose(6)];

== matlab function unreal_cosim/propPoses/Set Slalom Poses/Set White Slalom Pose 6/drift ==
  data: t input; pose input; driftPose output
function driftPose = drift(t,pose)
driftPose = toDriftedCoordinates(pose,t);

== matlab function unreal_cosim/propPoses/MATLAB Function ==
  data: manateePose input; obsPose output
function obsPose = getObsPose(manateePose)
d = 200;
pitch = -pi/6;
yaw = pi/6;
obsPose = [(manateePose(1) - d*cos(pitch)*cos(yaw)) (manateePose(2) - d*cos(pitch)*sin(yaw)) (manateePose(3) + d*sin(pitch)) 0 pitch yaw];

== matlab function unreal_cosim/propPoses/Set Gate1 Pose/MATLAB Function1 ==
  data: leftMountPose input; mountPose output
function mountPose = getMountPose(leftMountPose)

phi = leftMountPose(6) * pi / 180 + pi / 2;
xAdjust = 307 * cos(phi);
yAdjust = 307 * sin(phi);

mountPose = [(leftMountPose(1) + xAdjust) (leftMountPose(2) + yAdjust) leftMountPose(3) 0 0 leftMountPose(6)];

== matlab function unreal_cosim/propPoses/Set Slalom Poses/Set Red Slalom Pose 1/MATLAB Function ==
  data: mountedPose input; mountPose output; ground_Z parameter
function mountPose = getMountPose(mountedPose,ground_Z)

mountPose = [mountedPose(1) mountedPose(2) (10 - ground_Z) 0 0 mountedPose(6)];

== matlab function unreal_cosim/propPoses/Set Gate1 Pose/drift ==
  data: t input; pose input; driftPose output
function driftPose = drift(t,pose)
driftPose = toDriftedCoordinates(pose,t);

== matlab function unreal_cosim/propPoses/Set Slalom Poses/Set Red Slalom Pose 1/drift ==
  data: t input; pose input; driftPose output
function driftPose = drift(t,pose)
driftPose = toDriftedCoordinates(pose,t);

== matlab function unreal_cosim/propPoses/Set Slalom Poses/Set Red Slalom Pose 2/MATLAB Function ==
  data: mountedPose input; mountPose output; ground_Z parameter
function mountPose = getMountPose(mountedPose,ground_Z)

mountPose = [mountedPose(1) mountedPose(2) (10 - ground_Z) 0 0 mountedPose(6)];

== matlab function unreal_cosim/propPoses/Set Slalom Poses/Set Red Slalom Pose 2/drift ==
  data: t input; pose input; driftPose output
function driftPose = drift(t,pose)
driftPose = toDriftedCoordinates(pose,t);

== matlab function unreal_cosim/propPoses/Set Slalom Poses/Set Red Slalom Pose 3/MATLAB Function ==
  data: mountedPose input; mountPose output; ground_Z parameter
function mountPose = getMountPose(mountedPose,ground_Z)

mountPose = [mountedPose(1) mountedPose(2) (10 - ground_Z) 0 0 mountedPose(6)];

== matlab function unreal_cosim/propPoses/Set Slalom Poses/Set Red Slalom Pose 3/drift ==
  data: t input; pose input; driftPose output
function driftPose = drift(t,pose)
driftPose = toDriftedCoordinates(pose,t);

== matlab function unreal_cosim/propPoses/Set Slalom Poses/Set White Slalom Pose 1/MATLAB Function ==
  data: mountedPose input; mountPose output; ground_Z parameter
function mountPose = getMountPose(mountedPose,ground_Z)

mountPose = [mountedPose(1) mountedPose(2) (10 - ground_Z) 0 0 mountedPose(6)];

== matlab function unreal_cosim/propPoses/Set Slalom Poses/Set White Slalom Pose 1/drift ==
  data: t input; pose input; driftPose output
function driftPose = drift(t,pose)
driftPose = toDriftedCoordinates(pose,t);

== matlab function unreal_cosim/propPoses/Set Slalom Poses/Set White Slalom Pose 2/MATLAB Function ==
  data: mountedPose input; mountPose output; ground_Z parameter
function mountPose = getMountPose(mountedPose,ground_Z)

mountPose = [mountedPose(1) mountedPose(2) (10 - ground_Z) 0 0 mountedPose(6)];
